simulink model "Kirov_physics"  (R2024b)
settings: Solver=FixedStepDiscrete  StartTime=0.0  StopTime=inf  FixedStep=dt  RelTol=1e-3
undefined symbols (not defined in the file): accel_O, airspeed_bp, alpha_B, alpha_bp, alphaFull, alphaOff, b, battery_capacity_bp, battery_current_bp, battery_initial_capacity_mAh, battery_voltage_table, beta_bp, betaFull, betaOff, brake, brakes, c, channels, CLa, Clb, Clp, CLq, Clr, Cma, Cmq, Cnb, Cnp, Cnr, current_table, DiscIntNeverNeededParam, dt, ELEV_bp, elevator, f, flap, flaps, FLAPS_bp, gear, heightFadeStart, heightOff, hgt_0, Inertia_body, Inertia_load, kInduced, L_aileron, L_throttle, LAILE_bp, lat_0, lon_0, M_aile, M_body, M_elev, M_flap, M_front_gear, M_load, M_main_gear, M_prop, M_rudd, M_spoiler, minWingHeight ... (+36)
libraries: sm_lib x673, simulink x58, nesl_utility x51, simulink_extras x24, uavmavlinklib x12, instrumentlib x4, vrlib x3, aerolibfltsims x3, sharedtransform x3, eeGeneralControl x2, aerolibutil x2, AP_Connector x2
(part 4 of 6)

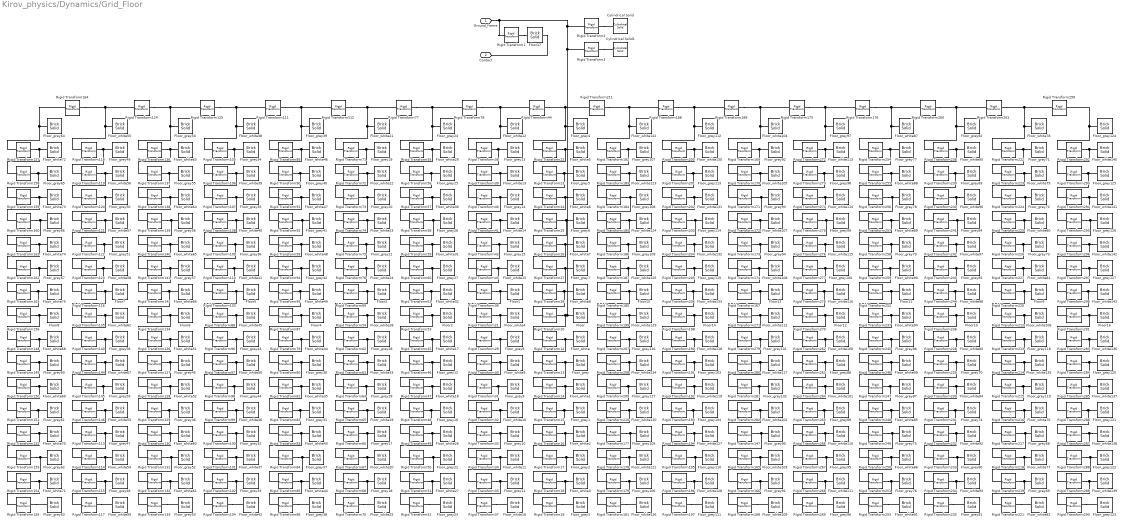
== system Kirov_physics/Dynamics/Grid_Floor ==
  Cylindrical Solid : sm_lib/Body Elements/Cylindrical Solid  CylinderRadius=0.2  CylinderRadiusUnits=m  CylinderLength=5  CylinderLengthUnits=m  ExportEntireGeometry=off  InertiaType=CalculateFromGeometry  BasedOnType=Density  Density=1000  DensityUnits=kg/m^3  Mass=1  MassUnits=kg  CenterOfMass=[0 0 0]  CenterOfMassUnits=m  MomentsOfInertia=[1 1 1]  MomentsOfInertiaUnits=kg*m^2  ProductsOfInertia=[0 0 0]  ProductsOfInertiaUnits=kg*m^2  GraphicType=FromGeometry  MarkerShape=Sphere  MarkerSize=10  GraphicVisPropType=SimpleVisualProperties  GraphicDiffuseColor=[1 0 0]  GraphicOpacity=1  GraphicSpecularColor=[0.5 0.5 0.5 1.0]  GraphicAmbientColor=[0.15 0.15 0.15 1.0]  GraphicEmissiveColor=[0.0 0.0 0.0 1.0]  GraphicShininess=75  DoExposeReferenceFrame=on  SerializedFrames=<Frames/>
  Cylindrical Solid1 : sm_lib/Body Elements/Cylindrical Solid  CylinderRadius=0.2  CylinderRadiusUnits=m  CylinderLength=5  CylinderLengthUnits=m  ExportEntireGeometry=off  InertiaType=CalculateFromGeometry  BasedOnType=Density  Density=1000  DensityUnits=kg/m^3  Mass=1  MassUnits=kg  CenterOfMass=[0 0 0]  CenterOfMassUnits=m  MomentsOfInertia=[1 1 1]  MomentsOfInertiaUnits=kg*m^2  ProductsOfInertia=[0 0 0]  ProductsOfInertiaUnits=kg*m^2  GraphicType=FromGeometry  MarkerShape=Sphere  MarkerSize=10  GraphicVisPropType=SimpleVisualProperties  GraphicDiffuseColor=[1 0 0]  GraphicOpacity=1  GraphicSpecularColor=[0.5 0.5 0.5 1.0]  GraphicAmbientColor=[0.15 0.15 0.15 1.0]  GraphicEmissiveColor=[0.0 0.0 0.0 1.0]  GraphicShininess=75  DoExposeReferenceFrame=on  SerializedFrames=<Frames/>
  Floor{,1..16} (17 alike) : sm_lib/Body Elements/Brick Solid  BrickDimensions=[10 10 0.1]  BrickDimensionsUnits=m  ExportEntireGeometry=off  InertiaType=PointMass  BasedOnType=Density  Density=1000  DensityUnits=kg/m^3  Mass=100  MassUnits=kg  CenterOfMass=[0 0 0]  CenterOfMassUnits=m  MomentsOfInertia=[1 1 1]  MomentsOfInertiaUnits=kg*m^2  ProductsOfInertia=[0 0 0]  ProductsOfInertiaUnits=kg*m^2  GraphicType=FromGeometry  MarkerShape=Sphere  MarkerSize=10  GraphicVisPropType=SimpleVisualProperties  GraphicDiffuseColor=[0.651 0.651 0.651]  GraphicOpacity=1  GraphicSpecularColor=[0.5 0.5 0.5 1.0]  GraphicAmbientColor=[0.15 0.15 0.15 1.0]  GraphicEmissiveColor=[0.0 0.0 0.0 1.0]  GraphicShininess=75  DoExposeReferenceFrame=on  SerializedFrames=<Frames/>
  Floor17 : sm_lib/Body Elements/Brick Solid  BrickDimensions=[2000 2000 0.1]  BrickDimensionsUnits=m  ExportEntireGeometry=on  InertiaType=PointMass  BasedOnType=Density  Density=1000  DensityUnits=kg/m^3  Mass=100  MassUnits=kg  CenterOfMass=[0 0 0]  CenterOfMassUnits=m  MomentsOfInertia=[1 1 1]  MomentsOfInertiaUnits=kg*m^2  ProductsOfInertia=[0 0 0]  ProductsOfInertiaUnits=kg*m^2  GraphicType=FromGeometry  MarkerShape=Sphere  MarkerSize=10  GraphicVisPropType=SimpleVisualProperties  GraphicDiffuseColor=[0.651 0.651 0.651]  GraphicOpacity=1  GraphicSpecularColor=[0.5 0.5 0.5 1.0]  GraphicAmbientColor=[0.15 0.15 0.15 1.0]  GraphicEmissiveColor=[0.0 0.0 0.0 1.0]  GraphicShininess=75  DoExposeReferenceFrame=on  SerializedFrames=<Frames/>
  Floor_grey{,1..127} (128 alike) : sm_lib/Body Elements/Brick Solid  BrickDimensions=[10 10 0.1]  BrickDimensionsUnits=m  ExportEntireGeometry=off  InertiaType=PointMass  BasedOnType=Density  Density=1000  DensityUnits=kg/m^3  Mass=100  MassUnits=kg  CenterOfMass=[0 0 0]  CenterOfMassUnits=m  MomentsOfInertia=[1 1 1]  MomentsOfInertiaUnits=kg*m^2  ProductsOfInertia=[0 0 0]  ProductsOfInertiaUnits=kg*m^2  GraphicType=FromGeometry  MarkerShape=Sphere  MarkerSize=10  GraphicVisPropType=SimpleVisualProperties  GraphicDiffuseColor=[0.651 0.651 0.651]  GraphicOpacity=1  GraphicSpecularColor=[0.5 0.5 0.5 1.0]  GraphicAmbientColor=[0.15 0.15 0.15 1.0]  GraphicEmissiveColor=[0.0 0.0 0.0 1.0]  GraphicShininess=75  DoExposeReferenceFrame=on  SerializedFrames=<Frames/>
  Floor_white{,1..143} (144 alike) : sm_lib/Body Elements/Brick Solid  BrickDimensions=[10 10 0.1]  BrickDimensionsUnits=m  ExportEntireGeometry=off  InertiaType=PointMass  BasedOnType=Density  Density=1000  DensityUnits=kg/m^3  Mass=100  MassUnits=kg  CenterOfMass=[0 0 0]  CenterOfMassUnits=m  MomentsOfInertia=[1 1 1]  MomentsOfInertiaUnits=kg*m^2  ProductsOfInertia=[0 0 0]  ProductsOfInertiaUnits=kg*m^2  GraphicType=FromGeometry  MarkerShape=Sphere  MarkerSize=10  GraphicVisPropType=SimpleVisualProperties  GraphicDiffuseColor=[1 1 1]  GraphicOpacity=1  GraphicSpecularColor=[0.5 0.5 0.5 1.0]  GraphicAmbientColor=[0.15 0.15 0.15 1.0]  GraphicEmissiveColor=[0.0 0.0 0.0 1.0]  GraphicShininess=75  DoExposeReferenceFrame=on  SerializedFrames=<Frames/>
  Rigid Transform1 : sm_lib/Frames and Transforms/Rigid Transform  RotationMethod=None  FollAlignAxisA=+X  BaseAlignAxisA=+Y  FollAlignAxisB=+Y  BaseAlignAxisB=+Z  RotationStandardAxis=+Z  RotationAngle=0  RotationAngleUnits=deg  RotationArbitraryAxis=[0 0 1]  RotationSequenceAxes=FollowerAxes  RotationSequence=XYX  RotationSequenceAngles=[0 0 0]  RotationSequenceAnglesUnits=deg  RotationMatrix=[1 0 0;0 1 0;0 0 1]  Quaternion=[1 0 0 0]  TranslationMethod=Cartesian  TranslationCartesianOffset=[0 0 0.005]  TranslationCartesianOffsetUnits=m  TranslationStandardAxis=+Z  TranslationStandardOffset=0  TranslationStandardOffsetUnits=m  TranslationROffset=0  TranslationROffsetUnits=m  TranslationThetaOffset=0  TranslationThetaOffsetUnits=deg  TranslationZOffset=0  TranslationZOffsetUnits=m
  Rigid Transform{12..43,45..76,79..110,113..123,126..163,165..174,177..187,190..210,212..259,262..298} (272 alike) : sm_lib/Frames and Transforms/Rigid Transform  RotationMethod=None  FollAlignAxisA=+X  BaseAlignAxisA=+Y  FollAlignAxisB=+Y  BaseAlignAxisB=+Z  RotationStandardAxis=+Z  RotationAngle=0  RotationAngleUnits=deg  RotationArbitraryAxis=[0 0 1]  RotationSequenceAxes=FollowerAxes  RotationSequence=XYX  RotationSequenceAngles=[0 0 0]  RotationSequenceAnglesUnits=deg  RotationMatrix=[1 0 0;0 1 0;0 0 1]  Quaternion=[1 0 0 0]  TranslationMethod=Cartesian  TranslationCartesianOffset=[10 0 0]  TranslationCartesianOffsetUnits=m  TranslationStandardAxis=+Z  TranslationStandardOffset=0  TranslationStandardOffsetUnits=m  TranslationROffset=0  TranslationROffsetUnits=m  TranslationThetaOffset=0  TranslationThetaOffsetUnits=deg  TranslationZOffset=0  TranslationZOffsetUnits=m
  Rigid Transform{44,77..78,111..112,124..125,164,175..176,188..189,211,260..261,299} (16 alike) : sm_lib/Frames and Transforms/Rigid Transform  RotationMethod=None  FollAlignAxisA=+X  BaseAlignAxisA=+Y  FollAlignAxisB=+Y  BaseAlignAxisB=+Z  RotationStandardAxis=+Z  RotationAngle=0  RotationAngleUnits=deg  RotationArbitraryAxis=[0 0 1]  RotationSequenceAxes=FollowerAxes  RotationSequence=XYX  RotationSequenceAngles=[0 0 0]  RotationSequenceAnglesUnits=deg  RotationMatrix=[1 0 0;0 1 0;0 0 1]  Quaternion=[1 0 0 0]  TranslationMethod=Cartesian  TranslationCartesianOffset=[0 10 0]  TranslationCartesianOffsetUnits=m  TranslationStandardAxis=+Z  TranslationStandardOffset=0  TranslationStandardOffsetUnits=m  TranslationROffset=0  TranslationROffsetUnits=m  TranslationThetaOffset=0  TranslationThetaOffsetUnits=deg  TranslationZOffset=0  TranslationZOffsetUnits=m
  Rigid Transform2 : sm_lib/Frames and Transforms/Rigid Transform  RotationMethod=None  FollAlignAxisA=+X  BaseAlignAxisA=+Y  FollAlignAxisB=+Y  BaseAlignAxisB=+Z  RotationStandardAxis=+Z  RotationAngle=0  RotationAngleUnits=deg  RotationArbitraryAxis=[0 0 1]  RotationSequenceAxes=FollowerAxes  RotationSequence=XYX  RotationSequenceAngles=[0 0 0]  RotationSequenceAnglesUnits=deg  RotationMatrix=[1 0 0;0 1 0;0 0 1]  Quaternion=[1 0 0 0]  TranslationMethod=Cartesian  TranslationCartesianOffset=[50 20 -2.5]  TranslationCartesianOffsetUnits=m  TranslationStandardAxis=+Z  TranslationStandardOffset=0  TranslationStandardOffsetUnits=m  TranslationROffset=0  TranslationROffsetUnits=m  TranslationThetaOffset=0  TranslationThetaOffsetUnits=deg  TranslationZOffset=0  TranslationZOffsetUnits=m
  Rigid Transform3 : sm_lib/Frames and Transforms/Rigid Transform  RotationMethod=None  FollAlignAxisA=+X  BaseAlignAxisA=+Y  FollAlignAxisB=+Y  BaseAlignAxisB=+Z  RotationStandardAxis=+Z  RotationAngle=0  RotationAngleUnits=deg  RotationArbitraryAxis=[0 0 1]  RotationSequenceAxes=FollowerAxes  RotationSequence=XYX  RotationSequenceAngles=[0 0 0]  RotationSequenceAnglesUnits=deg  RotationMatrix=[1 0 0;0 1 0;0 0 1]  Quaternion=[1 0 0 0]  TranslationMethod=Cartesian  TranslationCartesianOffset=[-50 20 -2.5]  TranslationCartesianOffsetUnits=m  TranslationStandardAxis=+Z  TranslationStandardOffset=0  TranslationStandardOffsetUnits=m  TranslationROffset=0  TranslationROffsetUnits=m  TranslationThetaOffset=0  TranslationThetaOffsetUnits=deg  TranslationZOffset=0  TranslationZOffsetUnits=m
  Ground_frame : PMIOPort  Side=Left
  Contact : PMIOPort  Port=2  Side=Right
  connections:
  Rigid Transform158/RConn1 -- Rigid Transform159/LConn1 -- Floor_grey65/RConn1
  Rigid Transform156/LConn1 -- Rigid Transform163/RConn1 -- Floor_white75/RConn1
  Rigid Transform168/RConn1 -- Floor_white109/RConn1
  Floor_white120/RConn1 -- Rigid Transform177/LConn1 -- Rigid Transform210/RConn1
  Rigid Transform198/LConn1 -- Rigid Transform206/RConn1 -- Floor_white133/RConn1
  Floor_white85/RConn1 -- Rigid Transform249/LConn1 -- Rigid Transform248/RConn1
  Rigid Transform244/LConn1 -- Rigid Transform243/RConn1 -- Floor_grey85/RConn1
  Rigid Transform245/RConn1 -- Rigid Transform246/LConn1 -- Floor_grey86/RConn1
  Floor_white122/RConn1 -- Rigid Transform211/RConn1 -- Rigid Transform188/LConn1 -- Rigid Transform182/LConn1
  Rigid Transform241/RConn1 -- Rigid Transform242/LConn1 -- Floor_grey84/RConn1
  Rigid Transform284/RConn1 -- Rigid Transform285/LConn1 -- Floor_grey120/RConn1
  Floor8/RConn1 -- Rigid Transform156/RConn1 -- Rigid Transform148/LConn1
  Floor_white93/RConn1 -- Rigid Transform235/LConn1 -- Rigid Transform234/RConn1
  Rigid Transform180/RConn1 -- Floor15/RConn1 -- Rigid Transform199/LConn1
  Rigid Transform282/LConn1 -- Rigid Transform281/RConn1 -- Floor_grey102/RConn1
  Rigid Transform127/RConn1 -- Rigid Transform128/LConn1 -- Floor_grey45/RConn1
  Rigid Transform243/LConn1 -- Floor_white97/RConn1 -- Rigid Transform242/RConn1
  Rigid Transform160/RConn1 -- Rigid Transform161/LConn1 -- Floor_grey66/RConn1
  Rigid Transform133/LConn1 -- Floor_white61/RConn1 -- Rigid Transform132/RConn1
  Rigid Transform257/LConn1 -- Rigid Transform256/RConn1 -- Floor_grey78/RConn1
  Rigid Transform123/LConn1 -- Rigid Transform122/RConn1 -- Floor_grey51/RConn1
  Rigid Transform295/LConn1 -- Floor_white141/RConn1 -- Rigid Transform294/RConn1
  Rigid Transform184/LConn1 -- Floor_white123/RConn1 -- Rigid Transform183/RConn1
  Rigid Transform120/RConn1 -- Rigid Transform121/LConn1 -- Floor_grey50/RConn1
  Rigid Transform226/LConn1 -- Floor_white80/RConn1 -- Rigid Transform225/RConn1
  Rigid Transform224/RConn1 -- Rigid Transform225/LConn1 -- Floor_grey72/RConn1
  Floor_white131/RConn1 -- Rigid Transform203/LConn1 -- Rigid Transform202/RConn1
  Rigid Transform152/LConn1 -- Rigid Transform151/RConn1 -- Floor_grey61/RConn1
  Floor_white65/RConn1 -- Rigid Transform141/LConn1 -- Rigid Transform140/RConn1
  Rigid Transform144/RConn1 -- Rigid Transform145/LConn1 -- Floor_white67/RConn1
  Rigid Transform197/RConn1 -- Floor_grey111/RConn1
  Rigid Transform179/LConn1 -- Floor_white121/RConn1 -- Rigid Transform178/RConn1
  Rigid Transform122/LConn1 -- Floor_white57/RConn1 -- Rigid Transform121/RConn1
  Rigid Transform52/LConn1 -- Floor_white27/RConn1 -- Rigid Transform51/RConn1
  Rigid Transform58/LConn1 -- Floor_white30/RConn1 -- Rigid Transform57/RConn1
  Rigid Transform283/RConn1 -- Rigid Transform284/LConn1 -- Floor_white136/RConn1
  Rigid Transform57/LConn1 -- Rigid Transform56/RConn1 -- Floor_grey25/RConn1
  Floor_white105/RConn1 -- Rigid Transform171/LConn1 -- Rigid Transform170/RConn1
  Rigid Transform201/LConn1 -- Rigid Transform200/RConn1 -- Floor_white130/RConn1
  Rigid Transform150/RConn1 -- Rigid Transform151/LConn1 -- Floor_white69/RConn1
  Rigid Transform181/RConn1 -- Floor_white126/RConn1
  Rigid Transform158/LConn1 -- Rigid Transform157/RConn1 -- Floor_white72/RConn1
  Rigid Transform256/LConn1 -- Floor_white88/RConn1 -- Rigid Transform255/RConn1
  Floor_white26/RConn1 -- Rigid Transform50/LConn1 -- Rigid Transform49/RConn1
  Rigid Transform163/LConn1 -- Rigid Transform162/RConn1 -- Floor_grey67/RConn1
  Rigid Transform70/RConn1 -- Floor_white25/RConn1
  Rigid Transform147/LConn1 -- Floor_white102/RConn1 -- Rigid Transform282/RConn1
  Rigid Transform201/RConn1 -- Rigid Transform202/LConn1 -- Floor_grey113/RConn1
  Rigid Transform277/RConn1 -- Rigid Transform278/LConn1 -- Floor_grey100/RConn1
  Rigid Transform175/RConn1 -- Rigid Transform176/LConn1 -- Rigid Transform272/LConn1 -- Floor_grey97/RConn1
  Rigid Transform211/LConn1 -- Rigid Transform44/RConn1 -- Floor_grey4/RConn1 -- Rigid Transform22/LConn1
  Rigid Transform196/LConn1 -- Rigid Transform195/RConn1 -- Floor_grey110/RConn1
  Rigid Transform183/LConn1 -- Rigid Transform182/RConn1 -- Floor_grey107/RConn1
  Rigid Transform136/RConn1 -- Rigid Transform137/LConn1 -- Floor_white63/RConn1
  Rigid Transform23/RConn1 -- Rigid Transform24/LConn1 -- Floor_grey5/RConn1
  Rigid Transform23/LConn1 -- Rigid Transform22/RConn1 -- Floor_white5/RConn1
  Rigid Transform14/LConn1 -- Rigid Transform13/RConn1 -- Floor_grey/RConn1
  Rigid Transform239/LConn1 -- Rigid Transform238/RConn1 -- Floor_white95/RConn1
  Rigid Transform194/LConn1 -- Rigid Transform193/RConn1 -- Floor_grey104/RConn1
  Rigid Transform138/LConn1 -- Rigid Transform137/RConn1 -- Floor_grey55/RConn1
  Rigid Transform191/LConn1 -- Rigid Transform190/RConn1 -- Floor_white118/RConn1
  Rigid Transform27/LConn1 -- Floor_white7/RConn1 -- Rigid Transform26/RConn1
  Rigid Transform269/RConn1 -- Floor_grey96/RConn1
  Floor_white60/RConn1 -- Rigid Transform131/LConn1 -- Rigid Transform130/RConn1
  Rigid Transform237/RConn1 -- Rigid Transform245/LConn1 -- Floor_white94/RConn1
  Rigid Transform43/RConn1 -- Rigid Transform36/LConn1 -- Floor_white15/RConn1
  Rigid Transform45/RConn1 -- Rigid Transform46/LConn1 -- Floor_white17/RConn1
  Rigid Transform13/LConn1 -- Rigid Transform12/RConn1 -- Floor_white/RConn1
  Rigid Transform78/RConn1 -- Rigid Transform38/LConn1 -- Floor_white12/RConn1 -- Rigid Transform44/LConn1
  Rigid Transform220/LConn1 -- Rigid Transform227/RConn1 -- Floor_white81/RConn1
  Rigid Transform134/RConn1 -- Floor6/RConn1 -- Rigid Transform126/LConn1
  Rigid Transform259/RConn1 -- Rigid Transform252/LConn1 -- Floor_white90/RConn1
  Floor_white14/RConn1 -- Rigid Transform42/LConn1 -- Rigid Transform41/RConn1
  Rigid Transform143/LConn1 -- Rigid Transform135/RConn1 -- Floor_white62/RConn1
  Rigid Transform294/LConn1 -- Rigid Transform293/RConn1 -- Floor_grey125/RConn1
  Rigid Transform279/LConn1 -- Rigid Transform271/RConn1 -- Floor_white112/RConn1
  Rigid Transform133/RConn1 -- Floor_grey53/RConn1
  Rigid Transform144/LConn1 -- Rigid Transform143/RConn1 -- Floor_grey58/RConn1
  Rigid Transform33/RConn1 -- Rigid Transform34/LConn1 -- Floor_grey10/RConn1
  Rigid Transform169/RConn1 -- Rigid Transform170/LConn1 -- Floor_grey92/RConn1
  Rigid Transform114/LConn1 -- Rigid Transform113/RConn1 -- Floor_grey47/RConn1
  Rigid Transform17/LConn1 -- Floor_white2/RConn1 -- Rigid Transform16/RConn1
  Rigid Transform164/LConn1 -- Floor_grey64/RConn1 -- Rigid Transform157/LConn1
  Rigid Transform25/RConn1 -- Rigid Transform26/LConn1 -- Floor_grey6/RConn1
  Rigid Transform209/LConn1 -- Rigid Transform208/RConn1 -- Floor_white134/RConn1
  Rigid Transform21/RConn1 -- Rigid Transform29/LConn1 -- Floor_white4/RConn1
  Rigid Transform14/RConn1 -- Rigid Transform15/LConn1 -- Floor_white1/RConn1
  Floor_white128/RConn1 -- Rigid Transform197/LConn1 -- Rigid Transform196/RConn1
  Rigid Transform140/LConn1 -- Rigid Transform139/RConn1 -- Floor_grey56/RConn1
  Rigid Transform42/RConn1 -- Rigid Transform43/LConn1 -- Floor_grey15/RConn1
  Floor_white10/RConn1 -- Rigid Transform33/LConn1 -- Rigid Transform32/RConn1
  Rigid Transform230/RConn1 -- Rigid Transform231/LConn1 -- Floor_white84/RConn1
  Floor_white142/RConn1 -- Rigid Transform297/LConn1 -- Rigid Transform296/RConn1
  Rigid Transform116/LConn1 -- Rigid Transform123/RConn1 -- Floor_white58/RConn1
  Rigid Transform67/LConn1 -- Rigid Transform66/RConn1 -- Floor_grey17/RConn1
  Rigid Transform192/RConn1 -- Rigid Transform193/LConn1 -- Floor_white119/RConn1
  Floor10/RConn1 -- Rigid Transform236/RConn1 -- Rigid Transform228/LConn1
  Rigid Transform213/LConn1 -- Rigid Transform212/RConn1 -- Floor_white106/RConn1
  Floor_white138/RConn1 -- Rigid Transform288/LConn1 -- Rigid Transform287/RConn1
  Floor_white73/RConn1 -- Rigid Transform160/LConn1 -- Rigid Transform159/RConn1
  Rigid Transform37/LConn1 -- Rigid Transform35/RConn1 -- Floor_grey11/RConn1
  Rigid Transform19/RConn1 -- Floor_grey3/RConn1
  Floor_white3/RConn1 -- Rigid Transform19/LConn1 -- Rigid Transform18/RConn1
  Rigid Transform139/LConn1 -- Floor_white64/RConn1 -- Rigid Transform138/RConn1
  Ground_frame/RConn1 -- Rigid Transform1/LConn1 -- Rigid Transform2/LConn1 -- Rigid Transform3/LConn1 -- Floor/RConn1 -- Rigid Transform20/RConn1 -- Rigid Transform12/LConn1
  Rigid Transform46/RConn1 -- Rigid Transform47/LConn1 -- Floor_grey12/RConn1
  Rigid Transform50/RConn1 -- Rigid Transform51/LConn1 -- Floor_grey22/RConn1
  Floor3/RConn1 -- Rigid Transform69/RConn1 -- Rigid Transform54/LConn1
  Rigid Transform31/RConn1 -- Rigid Transform32/LConn1 -- Floor_grey9/RConn1
  Rigid Transform60/RConn1 -- Rigid Transform61/LConn1 -- Floor_grey27/RConn1
  Rigid Transform232/LConn1 -- Rigid Transform231/RConn1 -- Floor_grey74/RConn1
  Rigid Transform280/LConn1 -- Rigid Transform279/RConn1 -- Floor_grey101/RConn1
  Rigid Transform219/RConn1 -- Rigid Transform221/LConn1 -- Floor_grey69/RConn1
  Rigid Transform298/RConn1 -- Rigid Transform291/LConn1 -- Floor_white143/RConn1
  Rigid Transform48/RConn1 -- Rigid Transform49/LConn1 -- Floor_grey16/RConn1
  Rigid Transform154/LConn1 -- Rigid Transform153/RConn1 -- Floor_grey62/RConn1
  Rigid Transform100/RConn1 -- Rigid Transform101/LConn1 -- Floor_grey32/RConn1
  Rigid Transform263/RConn1 -- Rigid Transform264/LConn1 -- Floor_grey88/RConn1
  Rigid Transform235/RConn1 -- Floor_grey81/RConn1
  Rigid Transform166/RConn1 -- Rigid Transform168/LConn1 -- Floor_grey91/RConn1
  Rigid Transform269/LConn1 -- Floor_white111/RConn1 -- Rigid Transform268/RConn1
  Floor_white20/RConn1 -- Rigid Transform68/LConn1 -- Rigid Transform67/RConn1
  Rigid Transform288/RConn1 -- Rigid Transform289/LConn1 -- Floor_grey122/RConn1
  Rigid Transform98/LConn1 -- Rigid Transform97/RConn1 -- Floor_white50/RConn1
  Rigid Transform62/LConn1 -- Rigid Transform54/RConn1 -- Floor_white28/RConn1
  Rigid Transform292/RConn1 -- Rigid Transform293/LConn1 -- Floor_white140/RConn1
  Floor14/RConn1 -- Rigid Transform198/RConn1 -- Rigid Transform190/LConn1
  Rigid Transform98/RConn1 -- Rigid Transform99/LConn1 -- Floor_grey44/RConn1
  Rigid Transform189/LConn1 -- Rigid Transform188/RConn1 -- Floor_grey112/RConn1 -- Rigid Transform200/LConn1
  Rigid Transform272/RConn1 -- Rigid Transform273/LConn1 -- Floor_white113/RConn1
  Rigid Transform65/LConn1 -- Rigid Transform64/RConn1 -- Floor_grey29/RConn1
  Rigid Transform131/RConn1 -- Rigid Transform132/LConn1 -- Floor_grey52/RConn1
  Rigid Transform125/RConn1 -- Rigid Transform111/LConn1 -- Rigid Transform105/LConn1 -- Floor_white38/RConn1
  Floor_white87/RConn1 -- Rigid Transform260/LConn1 -- Rigid Transform176/RConn1 -- Rigid Transform254/LConn1
  Rigid Transform169/LConn1 -- Rigid Transform189/RConn1 -- Rigid Transform175/LConn1 -- Floor_white104/RConn1
  Floor_white36/RConn1 -- Rigid Transform100/LConn1 -- Rigid Transform99/RConn1
  Rigid Transform95/LConn1 -- Rigid Transform94/RConn1 -- Floor_grey42/RConn1
  Rigid Transform149/LConn1 -- Rigid Transform148/RConn1 -- Floor_white68/RConn1
  Rigid Transform142/RConn1 -- Rigid Transform134/LConn1 -- Floor_white66/RConn1
  Rigid Transform18/LConn1 -- Rigid Transform17/RConn1 -- Floor_grey2/RConn1
  Rigid Transform41/LConn1 -- Rigid Transform40/RConn1 -- Floor_grey14/RConn1
  Floor13/RConn1 -- Rigid Transform167/RConn1 -- Rigid Transform271/LConn1
  Rigid Transform251/LConn1 -- Floor_white86/RConn1 -- Rigid Transform250/RConn1
  Rigid Transform113/LConn1 -- Floor_white53/RConn1 -- Rigid Transform146/RConn1
  Floor_white115/RConn1 -- Rigid Transform277/LConn1 -- Rigid Transform276/RConn1
  Rigid Transform181/LConn1 -- Rigid Transform179/RConn1 -- Floor_grey106/RConn1
  Floor_white31/RConn1 -- Rigid Transform60/LConn1 -- Rigid Transform59/RConn1
  Floor7/RConn1 -- Rigid Transform116/RConn1 -- Rigid Transform135/LConn1
  Floor_white56/RConn1 -- Rigid Transform120/LConn1 -- Rigid Transform119/RConn1
  Rigid Transform236/LConn1 -- Rigid Transform244/RConn1 -- Floor_white98/RConn1
  Floor_white79/RConn1 -- Rigid Transform224/LConn1 -- Rigid Transform223/RConn1
  Rigid Transform29/RConn1 -- Rigid Transform30/LConn1 -- Floor_grey8/RConn1
  Rigid Transform16/LConn1 -- Rigid Transform15/RConn1 -- Floor_grey1/RConn1
  Rigid Transform270/RConn1 -- Floor12/RConn1 -- Rigid Transform262/LConn1
  Rigid Transform174/LConn1 -- Rigid Transform173/RConn1 -- Floor_grey94/RConn1
  Rigid Transform92/RConn1 -- Rigid Transform93/LConn1 -- Floor_grey41/RConn1
  Rigid Transform286/RConn1 -- Rigid Transform287/LConn1 -- Floor_grey121/RConn1
  Rigid Transform55/RConn1 -- Rigid Transform56/LConn1 -- Floor_white29/RConn1
  Rigid Transform94/LConn1 -- Floor_white48/RConn1 -- Rigid Transform93/RConn1
  Rigid Transform275/LConn1 -- Floor_white114/RConn1 -- Rigid Transform274/RConn1
  Floor_white47/RConn1 -- Rigid Transform92/LConn1 -- Rigid Transform91/RConn1
  Rigid Transform117/RConn1 -- Floor_white59/RConn1
  Rigid Transform227/LConn1 -- Rigid Transform226/RConn1 -- Floor_grey73/RConn1
  Rigid Transform207/RConn1 -- Rigid Transform208/LConn1 -- Floor_grey116/RConn1
  Floor_white44/RConn1 -- Rigid Transform86/LConn1 -- Rigid Transform85/RConn1
  Rigid Transform63/LConn1 -- Rigid Transform62/RConn1 -- Floor_grey28/RConn1
  Rigid Transform78/LConn1 -- Rigid Transform77/RConn1 -- Rigid Transform55/LConn1 -- Floor_grey24/RConn1
  Rigid Transform299/RConn1 -- Rigid Transform292/LConn1 -- Floor_grey124/RConn1
  Rigid Transform229/LConn1 -- Rigid Transform228/RConn1 -- Floor_white83/RConn1
  Rigid Transform90/RConn1 -- Rigid Transform91/LConn1 -- Floor_grey40/RConn1
  Rigid Transform253/LConn1 -- Rigid Transform251/RConn1 -- Floor_grey76/RConn1
  Rigid Transform141/RConn1 -- Rigid Transform142/LConn1 -- Floor_grey57/RConn1
  Rigid Transform286/LConn1 -- Rigid Transform285/RConn1 -- Floor_white137/RConn1
  Rigid Transform262/RConn1 -- Rigid Transform263/LConn1 -- Floor_white100/RConn1
  Rigid Transform129/RConn1 -- Rigid Transform130/LConn1 -- Floor_grey46/RConn1
  Rigid Transform69/LConn1 -- Rigid Transform76/RConn1 -- Floor_white24/RConn1
  Rigid Transform217/LConn1 -- Floor_white76/RConn1 -- Rigid Transform216/RConn1
  Rigid Transform233/LConn1 -- Floor_white92/RConn1 -- Rigid Transform232/RConn1
  Floor_white103/RConn1 -- Rigid Transform166/LConn1 -- Rigid Transform165/RConn1
  Rigid Transform234/LConn1 -- Rigid Transform233/RConn1 -- Floor_grey80/RConn1
  Rigid Transform115/RConn1 -- Rigid Transform117/LConn1 -- Floor_grey48/RConn1
  Rigid Transform173/LConn1 -- Floor_white107/RConn1 -- Rigid Transform172/RConn1
  Rigid Transform214/LConn1 -- Rigid Transform213/RConn1 -- Floor_grey118/RConn1
  Rigid Transform36/RConn1 -- Floor1/RConn1 -- Rigid Transform21/LConn1
  Floor_white54/RConn1 -- Rigid Transform115/LConn1 -- Rigid Transform114/RConn1
  Rigid Transform146/LConn1 -- Rigid Transform145/RConn1 -- Floor_grey59/RConn1
  Rigid Transform247/LConn1 -- Rigid Transform246/RConn1 -- Floor_white99/RConn1
  Rigid Transform71/RConn1 -- Rigid Transform72/LConn1 -- Floor_grey19/RConn1
  Rigid Transform103/RConn1 -- Floor5/RConn1 -- Rigid Transform88/LConn1
  Rigid Transform153/LConn1 -- Floor_white70/RConn1 -- Rigid Transform152/RConn1
  Rigid Transform81/LConn1 -- Rigid Transform80/RConn1 -- Floor_grey30/RConn1
  Rigid Transform37/RConn1 -- Floor_white16/RConn1
  Rigid Transform35/LConn1 -- Floor_white11/RConn1 -- Rigid Transform34/RConn1
  Rigid Transform150/LConn1 -- Rigid Transform149/RConn1 -- Floor_grey60/RConn1
  Floor_white40/RConn1 -- Rigid Transform109/LConn1 -- Rigid Transform108/RConn1
  Rigid Transform102/LConn1 -- Floor_white37/RConn1 -- Rigid Transform101/RConn1
  Rigid Transform31/LConn1 -- Rigid Transform30/RConn1 -- Floor_white9/RConn1
  Rigid Transform52/RConn1 -- Floor_grey23/RConn1
  Rigid Transform205/LConn1 -- Floor_white132/RConn1 -- Rigid Transform204/RConn1
  Rigid Transform278/RConn1 -- Rigid Transform270/LConn1 -- Floor_white116/RConn1
  Rigid Transform276/LConn1 -- Rigid Transform275/RConn1 -- Floor_grey99/RConn1
  Rigid Transform104/LConn1 -- Rigid Transform102/RConn1 -- Floor_grey33/RConn1
  Rigid Transform155/RConn1 -- Floor_grey63/RConn1
  Rigid Transform89/LConn1 -- Rigid Transform112/LConn1 -- Rigid Transform111/RConn1 -- Floor_grey39/RConn1
  Rigid Transform255/LConn1 -- Rigid Transform254/RConn1 -- Floor_grey77/RConn1
  Rigid Transform177/RConn1 -- Rigid Transform178/LConn1 -- Floor_grey105/RConn1
  Rigid Transform83/LConn1 -- Rigid Transform82/RConn1 -- Floor_grey31/RConn1
  Rigid Transform186/RConn1 -- Rigid Transform187/LConn1 -- Floor_grey109/RConn1
  Rigid Transform39/LConn1 -- Rigid Transform38/RConn1 -- Floor_grey13/RConn1
  Rigid Transform107/LConn1 -- Floor_white39/RConn1 -- Rigid Transform106/RConn1
  Rigid Transform73/RConn1 -- Rigid Transform74/LConn1 -- Floor_grey20/RConn1
  Floor_white6/RConn1 -- Rigid Transform25/LConn1 -- Rigid Transform24/RConn1
  Rigid Transform68/RConn1 -- Rigid Transform70/LConn1 -- Floor_grey18/RConn1
  Rigid Transform104/RConn1 -- Floor_white42/RConn1
  Rigid Transform63/RConn1 -- Rigid Transform64/LConn1 -- Floor_white33/RConn1
  Rigid Transform40/LConn1 -- Floor_white13/RConn1 -- Rigid Transform39/RConn1
  Floor_white77/RConn1 -- Rigid Transform219/LConn1 -- Rigid Transform218/RConn1
  Rigid Transform165/LConn1 -- Rigid Transform147/RConn1 -- Floor_grey90/RConn1
  Rigid Transform265/RConn1 -- Rigid Transform266/LConn1 -- Floor_grey89/RConn1
  Rigid Transform296/LConn1 -- Rigid Transform295/RConn1 -- Floor_grey126/RConn1
  Rigid Transform106/LConn1 -- Rigid Transform105/RConn1 -- Floor_grey34/RConn1
  Rigid Transform206/LConn1 -- Rigid Transform205/RConn1 -- Floor_grey115/RConn1
  Rigid Transform164/RConn1 -- Rigid Transform124/LConn1 -- Floor_white55/RConn1 -- Rigid Transform118/LConn1
  Rigid Transform66/LConn1 -- Floor_white19/RConn1 -- Rigid Transform65/RConn1
  Rigid Transform124/RConn1 -- Rigid Transform125/LConn1 -- Rigid Transform136/LConn1 -- Floor_grey54/RConn1
  Rigid Transform280/RConn1 -- Rigid Transform281/LConn1 -- Floor_white117/RConn1
  Rigid Transform76/LConn1 -- Rigid Transform75/RConn1 -- Floor_grey21/RConn1
  Rigid Transform218/LConn1 -- Rigid Transform217/RConn1 -- Floor_grey68/RConn1
  Rigid Transform108/LConn1 -- Rigid Transform107/RConn1 -- Floor_grey35/RConn1
  Rigid Transform61/RConn1 -- Rigid Transform53/LConn1 -- Floor_white32/RConn1
  Rigid Transform192/LConn1 -- Rigid Transform191/RConn1 -- Floor_grey103/RConn1
  Rigid Transform20/LConn1 -- Rigid Transform28/RConn1 -- Floor_white8/RConn1
  Rigid Transform214/RConn1 -- Rigid Transform215/LConn1 -- Floor_white135/RConn1
  Floor_white110/RConn1 -- Rigid Transform267/LConn1 -- Rigid Transform266/RConn1
  Rigid Transform59/LConn1 -- Rigid Transform58/RConn1 -- Floor_grey26/RConn1
  Rigid Transform87/LConn1 -- Rigid Transform95/RConn1 -- Floor_white49/RConn1
  Rigid Transform221/RConn1 -- Floor_white82/RConn1
  Rigid Transform86/RConn1 -- Floor_grey38/RConn1
  Floor9/RConn1 -- Rigid Transform220/RConn1 -- Rigid Transform212/LConn1
  Floor_white124/RConn1 -- Rigid Transform186/LConn1 -- Rigid Transform185/RConn1
  Rigid Transform185/LConn1 -- Rigid Transform184/RConn1 -- Floor_grey108/RConn1
  Rigid Transform48/LConn1 -- Rigid Transform47/RConn1 -- Floor_white18/RConn1
  Rigid Transform167/LConn1 -- Rigid Transform174/RConn1 -- Floor_white108/RConn1
  Rigid Transform75/LConn1 -- Floor_white23/RConn1 -- Rigid Transform74/RConn1
  Rigid Transform239/RConn1 -- Rigid Transform240/LConn1 -- Floor_grey83/RConn1
  Rigid Transform203/RConn1 -- Rigid Transform204/LConn1 -- Floor_grey114/RConn1
  Rigid Transform195/LConn1 -- Floor_white127/RConn1 -- Rigid Transform194/RConn1
  Rigid Transform258/RConn1 -- Rigid Transform259/LConn1 -- Floor_grey79/RConn1
  Rigid Transform290/LConn1 -- Floor_white139/RConn1 -- Rigid Transform289/RConn1
  Rigid Transform85/LConn1 -- Rigid Transform84/RConn1 -- Floor_grey37/RConn1
  Rigid Transform249/RConn1 -- Rigid Transform250/LConn1 -- Floor_grey75/RConn1
  Rigid Transform110/RConn1 -- Rigid Transform103/LConn1 -- Floor_white41/RConn1
  Rigid Transform253/RConn1 -- Floor_white91/RConn1
  Rigid Transform162/LConn1 -- Floor_white74/RConn1 -- Rigid Transform161/RConn1
  Rigid Transform216/LConn1 -- Rigid Transform215/RConn1 -- Floor_grey119/RConn1
  Rigid Transform81/RConn1 -- Rigid Transform82/LConn1 -- Floor_white35/RConn1
  Rigid Transform252/RConn1 -- Floor11/RConn1 -- Rigid Transform237/LConn1
  Rigid Transform291/RConn1 -- Floor16/RConn1 -- Rigid Transform283/LConn1
  Rigid Transform187/RConn1 -- Rigid Transform180/LConn1 -- Floor_white125/RConn1
  Rigid Transform84/LConn1 -- Floor_white43/RConn1 -- Rigid Transform83/RConn1
  Rigid Transform129/LConn1 -- Rigid Transform128/RConn1 -- Floor_white52/RConn1
  Rigid Transform238/LConn1 -- Rigid Transform261/LConn1 -- Rigid Transform260/RConn1 -- Floor_grey82/RConn1
  Rigid Transform230/LConn1 -- Rigid Transform229/RConn1 -- Floor_grey70/RConn1
  Floor_white89/RConn1 -- Rigid Transform258/LConn1 -- Rigid Transform257/RConn1
  Floor_white22/RConn1 -- Rigid Transform73/LConn1 -- Rigid Transform72/RConn1
  Rigid Transform222/RConn1 -- Rigid Transform223/LConn1 -- Floor_grey71/RConn1
  Floor_white71/RConn1 -- Rigid Transform155/LConn1 -- Rigid Transform154/RConn1
  Rigid Transform109/RConn1 -- Rigid Transform110/LConn1 -- Floor_grey36/RConn1
  Rigid Transform90/LConn1 -- Rigid Transform89/RConn1 -- Floor_white46/RConn1
  Rigid Transform126/RConn1 -- Rigid Transform127/LConn1 -- Floor_white51/RConn1
  Rigid Transform88/RConn1 -- Rigid Transform96/LConn1 -- Floor_white45/RConn1
  Rigid Transform274/LConn1 -- Rigid Transform273/RConn1 -- Floor_grey98/RConn1
  Rigid Transform267/RConn1 -- Rigid Transform268/LConn1 -- Floor_grey95/RConn1
  Rigid Transform80/LConn1 -- Rigid Transform79/RConn1 -- Floor_white34/RConn1
  Rigid Transform297/RConn1 -- Rigid Transform298/LConn1 -- Floor_grey127/RConn1
  Rigid Transform118/RConn1 -- Rigid Transform119/LConn1 -- Floor_grey49/RConn1
  Rigid Transform53/RConn1 -- Floor2/RConn1 -- Rigid Transform45/LConn1
  Rigid Transform299/LConn1 -- Floor_white78/RConn1 -- Rigid Transform222/LConn1 -- Rigid Transform261/RConn1
  Floor4/RConn1 -- Rigid Transform87/RConn1 -- Rigid Transform79/LConn1
  Rigid Transform247/RConn1 -- Rigid Transform248/LConn1 -- Floor_grey87/RConn1
  Rigid Transform265/LConn1 -- Rigid Transform264/RConn1 -- Floor_white101/RConn1
  Rigid Transform171/RConn1 -- Rigid Transform172/LConn1 -- Floor_grey93/RConn1
  Rigid Transform290/RConn1 -- Floor_grey123/RConn1
  Rigid Transform199/RConn1 -- Rigid Transform207/LConn1 -- Floor_white129/RConn1
  Rigid Transform112/RConn1 -- Floor_white21/RConn1 -- Rigid Transform71/LConn1 -- Rigid Transform77/LConn1
  Floor_white96/RConn1 -- Rigid Transform241/LConn1 -- Rigid Transform240/RConn1
  Rigid Transform209/RConn1 -- Rigid Transform210/LConn1 -- Floor_grey117/RConn1
  Rigid Transform96/RConn1 -- Rigid Transform97/LConn1 -- Floor_grey43/RConn1
  Rigid Transform28/LConn1 -- Rigid Transform27/RConn1 -- Floor_grey7/RConn1
  Floor17/LConn1 -- Contact/RConn1
  Rigid Transform1/RConn1 -- Floor17/RConn1
  Rigid Transform2/RConn1 -- Cylindrical Solid/RConn1
  Rigid Transform3/RConn1 -- Cylindrical Solid1/RConn1

== system Kirov_physics/Dynamics/Subsystem ==
  Mechanism Configuration : sm_lib/Utilities/Mechanism Configuration  UniformGravity=Constant  GravityVector=[0 0 -9.80665]  GravityVectorUnits=m/s^2  LinearizationDelta=0.001  JointModeTransitionNonlinearIterations=2
  Rigid Transform : sm_lib/Frames and Transforms/Rigid Transform  RotationMethod=StandardAxis  FollAlignAxisA=+X  BaseAlignAxisA=+Y  FollAlignAxisB=+Y  BaseAlignAxisB=+Z  RotationStandardAxis=+X  RotationAngle=180  RotationAngleUnits=deg  RotationArbitraryAxis=[0 0 1]  RotationSequenceAxes=FollowerAxes  RotationSequence=XYX  RotationSequenceAngles=[0 0 0]  RotationSequenceAnglesUnits=deg  RotationMatrix=[1 0 0;0 1 0;0 0 1]  Quaternion=[1 0 0 0]  TranslationMethod=None  TranslationCartesianOffset=[0 0 0]  TranslationCartesianOffsetUnits=m  TranslationStandardAxis=+Z  TranslationStandardOffset=0  TranslationStandardOffsetUnits=m  TranslationROffset=0  TranslationROffsetUnits=m  TranslationThetaOffset=0  TranslationThetaOffsetUnits=deg  TranslationZOffset=0  TranslationZOffsetUnits=m
  Solver Configuration : nesl_utility/Solver Configuration  PhysicalDomain=network_engine_domain  SubClassName=solver  LeftPortType=input  RightPortType=generic  Tones=[]  Harmonics=[]  SimulateNoise=off  Profile=off  UseLocalSampling=off  EnableSwitchedLinearOptims=on  FrequencyDomain=off  UseCCode=off  RelTol=0.001  AbsTol=0.001  MinStep=1e-09  ToWorkspace=off  RevertToSquareIcSolve=off  NumHomotopyIterations=100  PhasorMode=off  PhasorModeNumHarmonics=1  ConsistencySolver=NEWTON_XTOL_AFTER_FTOL  IndexReductionMethod=DerivativeReplacement  DoDC=off  ResidualTolerance=1e-09  ConsistencyTolSource=GLOBAL  ConsistencyAbsTol=0.001  ConsistencyRelTol=0.001  ConsistencyTolFactor=0.001  UseLocalSolver=off  LocalSolverChoice=NE_BACKWARD_EULER_ADVANCER  ResolveIndetEquations=on  FunctionEvalNumThread=1  LocalSolverSampleTime=0.001  DoFixedCost=off  MaxNonlinIter=3  MaxModeIter=2  ComputeImpulses=off  ImpulseIterations=2  LinearAlgebra=auto  LinearAlgebraNumThread=0  EquationFormulation=NE_TIME_EF  DelaysMemoryBudget=1024  AutomaticFiltering=on  FilteringTimeConstant=0.001  PartitionStorageMethod=AS_NEEDED  PartitionMemoryBudget=1024  PartitionMethod=ROBUST  MultibodyUseLocalSolver=on  MultibodyLocalSolverChoice=ODE2  MultibodyLocalSolverSampleTime=0.001
  World Frame : sm_lib/Frames and Transforms/World Frame
  NED : PMIOPort  Side=Right
  connections:
  Rigid Transform/RConn1 -- NED/RConn1
  Mechanism Configuration/RConn1 -- Rigid Transform/LConn1 -- World Frame/RConn1 -- Solver Configuration/RConn1

== system Kirov_physics/Dynamics/Subsystem1 ==
  surface_input(deg) : Inport
  Degrees to Radians : simulink_extras/Transformations/Degrees to Radians
  Discrete Derivative : simulink/Quick Insert/Discrete/Discrete Derivative  gainval=1.0  ICPrevScaledInput=0.0  OutMin=[]  OutMax=[]  OutDataType=fixdt(1, 16)  OutScaling=2^-10  DoSatur=off
  Discrete Derivative1 : simulink/Quick Insert/Discrete/Discrete Derivative  gainval=1.0  ICPrevScaledInput=0.0  OutMin=[]  OutMax=[]  OutDataType=fixdt(1, 16)  OutScaling=2^-10  DoSatur=off
  Simulink-PS Converter : nesl_utility/Simulink-PS Converter  PhysicalDomain=network_engine_domain  SubClassName=ps_input  LeftPortType=input  RightPortType=output  PseudoPeriodic=off  Frequencies=[]  NoiseDistribution=none  NoiseParameters=[]  Unit=rad  AffineConversion=off  FilteringAndDerivatives=provide  SimscapeFilterOrder=1  InputFilterTimeConstant=0.001  UdotUserProvided=2
  surface_output : PMIOPort  Side=Right
  wires:
  surface_input(deg)/1 -> Degrees to Radians/1
  Discrete Derivative/1 -> Discrete Derivative1/1, Simulink-PS Converter/2
  Discrete Derivative1/1 -> Simulink-PS Converter/3
  Degrees to Radians/1 -> Discrete Derivative/1, Simulink-PS Converter/1
  connections:
  Simulink-PS Converter/RConn1 -- surface_output/RConn1

== system Kirov_physics/Dynamics/Subsystem10 ==
  torque_input(Nm) : Inport
  Discrete Derivative : simulink/Quick Insert/Discrete/Discrete Derivative  gainval=1.0  ICPrevScaledInput=0.0  OutMin=[]  OutMax=[]  OutDataType=fixdt(1, 16)  OutScaling=2^-10  DoSatur=off
  Discrete Derivative1 : simulink/Quick Insert/Discrete/Discrete Derivative  gainval=1.0  ICPrevScaledInput=0.0  OutMin=[]  OutMax=[]  OutDataType=fixdt(1, 16)  OutScaling=2^-10  DoSatur=off
  Simulink-PS Converter : nesl_utility/Simulink-PS Converter  PhysicalDomain=network_engine_domain  SubClassName=ps_input  LeftPortType=input  RightPortType=output  PseudoPeriodic=off  Frequencies=[]  NoiseDistribution=none  NoiseParameters=[]  Unit=N*m  AffineConversion=off  FilteringAndDerivatives=provide  SimscapeFilterOrder=1  InputFilterTimeConstant=0.001  UdotUserProvided=2
  torque_output : PMIOPort  Side=Right
  wires:
  Discrete Derivative1/1 -> Simulink-PS Converter/3
  Discrete Derivative/1 -> Simulink-PS Converter/2, Discrete Derivative1/1
  torque_input(Nm)/1 -> Simulink-PS Converter/1, Discrete Derivative/1
  connections:
  Simulink-PS Converter/RConn1 -- torque_output/RConn1

== system Kirov_physics/Dynamics/Subsystem11 ==
  torque_input(Nm) : Inport
  Discrete Derivative : simulink/Quick Insert/Discrete/Discrete Derivative  gainval=1.0  ICPrevScaledInput=0.0  OutMin=[]  OutMax=[]  OutDataType=fixdt(1, 16)  OutScaling=2^-10  DoSatur=off
  Discrete Derivative1 : simulink/Quick Insert/Discrete/Discrete Derivative  gainval=1.0  ICPrevScaledInput=0.0  OutMin=[]  OutMax=[]  OutDataType=fixdt(1, 16)  OutScaling=2^-10  DoSatur=off
  Simulink-PS Converter : nesl_utility/Simulink-PS Converter  PhysicalDomain=network_engine_domain  SubClassName=ps_input  LeftPortType=input  RightPortType=output  PseudoPeriodic=off  Frequencies=[]  NoiseDistribution=none  NoiseParameters=[]  Unit=N*m  AffineConversion=off  FilteringAndDerivatives=provide  SimscapeFilterOrder=1  InputFilterTimeConstant=0.001  UdotUserProvided=2
  torque_output : PMIOPort  Side=Right
  wires:
  torque_input(Nm)/1 -> Discrete Derivative/1, Simulink-PS Converter/1
  Discrete Derivative/1 -> Discrete Derivative1/1, Simulink-PS Converter/2
  Discrete Derivative1/1 -> Simulink-PS Converter/3
  connections:
  Simulink-PS Converter/RConn1 -- torque_output/RConn1

== system Kirov_physics/Dynamics/Subsystem12 ==
  torque_input(Nm) : Inport
  Discrete Derivative : simulink/Quick Insert/Discrete/Discrete Derivative  gainval=1.0  ICPrevScaledInput=0.0  OutMin=[]  OutMax=[]  OutDataType=fixdt(1, 16)  OutScaling=2^-10  DoSatur=off
  Discrete Derivative1 : simulink/Quick Insert/Discrete/Discrete Derivative  gainval=1.0  ICPrevScaledInput=0.0  OutMin=[]  OutMax=[]  OutDataType=fixdt(1, 16)  OutScaling=2^-10  DoSatur=off
  Simulink-PS Converter : nesl_utility/Simulink-PS Converter  PhysicalDomain=network_engine_domain  SubClassName=ps_input  LeftPortType=input  RightPortType=output  PseudoPeriodic=off  Frequencies=[]  NoiseDistribution=none  NoiseParameters=[]  Unit=N*m  AffineConversion=off  FilteringAndDerivatives=provide  SimscapeFilterOrder=1  InputFilterTimeConstant=0.001  UdotUserProvided=2
  torque_output : PMIOPort  Side=Right
  wires:
  Discrete Derivative1/1 -> Simulink-PS Converter/3
  Discrete Derivative/1 -> Simulink-PS Converter/2, Discrete Derivative1/1
  torque_input(Nm)/1 -> Simulink-PS Converter/1, Discrete Derivative/1
  connections:
  Simulink-PS Converter/RConn1 -- torque_output/RConn1

== system Kirov_physics/Dynamics/Subsystem13 ==
  flap_input : Inport
  Degrees to Radians : simulink_extras/Transformations/Degrees to Radians
  Gain2 : Gain  Gain=441.5/1000
  Gain3 : Gain  Gain=441.5/1000
  Subsystem13 : Subsystem
  Subsystem14 : Subsystem
  Subsystem15 : Subsystem
  dx : Lookup_n-D  NumberOfTableDimensions=1  BreakpointsForDimension1=[0, 1, 2]  BeginIndexSearchUsingPreviousIndexResult=on  Table=[0, -0.08819099, -0.21471805,]  InterpMethod=Linear Lagrange  DiagnosticForOutOfRangeInput=Error  InternalRulePriority=Speed  RndMeth=Simplest
  dz : Lookup_n-D  NumberOfTableDimensions=1  BreakpointsForDimension1=[0, 1, 2]  BeginIndexSearchUsingPreviousIndexResult=on  Table=[0, -0.15522630, -0.34229435]  InterpMethod=Linear Lagrange  DiagnosticForOutOfRangeInput=Error  InternalRulePriority=Speed  RndMeth=Simplest
  theta : Lookup_n-D  NumberOfTableDimensions=1  BreakpointsForDimension1=[0, 1, 2]  BeginIndexSearchUsingPreviousIndexResult=on  Table=[0, -13.24214507, -29.45123844]  InterpMethod=Linear Lagrange  DiagnosticForOutOfRangeInput=Error  InternalRulePriority=Speed  RndMeth=Simplest
  delta_x : PMIOPort  Side=Right
  delta_y : PMIOPort  Port=2  Side=Right
  rot_z : PMIOPort  Port=3  Side=Right
  wires:
  dz/1 -> Gain3/1
  Gain2/1 -> Subsystem14/1(surface_input)
  Gain3/1 -> Subsystem13/1(surface_input)
  dx/1 -> Gain2/1
  Degrees to Radians/1 -> Subsystem15/1(surface_input)
  theta/1 -> Degrees to Radians/1
  flap_input/1 -> dz/1, dx/1, theta/1
  connections:
  rot_z/RConn1 -- Subsystem15/RConn1
  Subsystem13/RConn1 -- delta_y/RConn1
  Subsystem14/RConn1 -- delta_x/RConn1

== system Kirov_physics/Dynamics/Subsystem14 ==
  surface_input(deg) : Inport
  Degrees to Radians : simulink_extras/Transformations/Degrees to Radians
  Discrete Derivative : simulink/Quick Insert/Discrete/Discrete Derivative  gainval=1.0  ICPrevScaledInput=0.0  OutMin=[]  OutMax=[]  OutDataType=fixdt(1, 16)  OutScaling=2^-10  DoSatur=off
  Discrete Derivative1 : simulink/Quick Insert/Discrete/Discrete Derivative  gainval=1.0  ICPrevScaledInput=0.0  OutMin=[]  OutMax=[]  OutDataType=fixdt(1, 16)  OutScaling=2^-10  DoSatur=off
  Simulink-PS Converter : nesl_utility/Simulink-PS Converter  PhysicalDomain=network_engine_domain  SubClassName=ps_input  LeftPortType=input  RightPortType=output  PseudoPeriodic=off  Frequencies=[]  NoiseDistribution=none  NoiseParameters=[]  Unit=rad  AffineConversion=off  FilteringAndDerivatives=provide  SimscapeFilterOrder=1  InputFilterTimeConstant=0.001  UdotUserProvided=2
  surface_output : PMIOPort  Side=Right
  wires:
  surface_input(deg)/1 -> Degrees to Radians/1
  Discrete Derivative/1 -> Discrete Derivative1/1, Simulink-PS Converter/2
  Discrete Derivative1/1 -> Simulink-PS Converter/3
  Degrees to Radians/1 -> Discrete Derivative/1, Simulink-PS Converter/1
  connections:
  Simulink-PS Converter/RConn1 -- surface_output/RConn1

== system Kirov_physics/Dynamics/Subsystem15 ==
  surface_input(deg) : Inport
  Degrees to Radians : simulink_extras/Transformations/Degrees to Radians
  Discrete Derivative : simulink/Quick Insert/Discrete/Discrete Derivative  gainval=1.0  ICPrevScaledInput=0.0  OutMin=[]  OutMax=[]  OutDataType=fixdt(1, 16)  OutScaling=2^-10  DoSatur=off
  Discrete Derivative1 : simulink/Quick Insert/Discrete/Discrete Derivative  gainval=1.0  ICPrevScaledInput=0.0  OutMin=[]  OutMax=[]  OutDataType=fixdt(1, 16)  OutScaling=2^-10  DoSatur=off
  Simulink-PS Converter : nesl_utility/Simulink-PS Converter  PhysicalDomain=network_engine_domain  SubClassName=ps_input  LeftPortType=input  RightPortType=output  PseudoPeriodic=off  Frequencies=[]  NoiseDistribution=none  NoiseParameters=[]  Unit=rad  AffineConversion=off  FilteringAndDerivatives=provide  SimscapeFilterOrder=1  InputFilterTimeConstant=0.001  UdotUserProvided=2
  surface_output : PMIOPort  Side=Right
  wires:
  Degrees to Radians/1 -> Simulink-PS Converter/1, Discrete Derivative/1
  Discrete Derivative1/1 -> Simulink-PS Converter/3
  Discrete Derivative/1 -> Simulink-PS Converter/2, Discrete Derivative1/1
  surface_input(deg)/1 -> Degrees to Radians/1
  connections:
  Simulink-PS Converter/RConn1 -- surface_output/RConn1

== system Kirov_physics/Dynamics/Subsystem16 ==
  flap_input : Inport
  Degrees to Radians : simulink_extras/Transformations/Degrees to Radians
  Gain2 : Gain  Gain=441.5/1000
  Gain3 : Gain  Gain=441.5/1000
  Subsystem13 : Subsystem
  Subsystem14 : Subsystem
  Subsystem15 : Subsystem
  dx : Lookup_n-D  NumberOfTableDimensions=1  BreakpointsForDimension1=[0, 1, 2]  BeginIndexSearchUsingPreviousIndexResult=on  Table=[0, -0.08819099, -0.21471805,]  InterpMethod=Linear Lagrange  DiagnosticForOutOfRangeInput=Error  InternalRulePriority=Speed  RndMeth=Simplest
  dz : Lookup_n-D  NumberOfTableDimensions=1  BreakpointsForDimension1=[0, 1, 2]  BeginIndexSearchUsingPreviousIndexResult=on  Table=[0, -0.15522630, -0.34229435]  InterpMethod=Linear Lagrange  DiagnosticForOutOfRangeInput=Error  InternalRulePriority=Speed  RndMeth=Simplest
  theta : Lookup_n-D  NumberOfTableDimensions=1  BreakpointsForDimension1=[0, 1, 2]  BeginIndexSearchUsingPreviousIndexResult=on  Table=[0, -13.24214507, -29.45123844]  InterpMethod=Linear Lagrange  DiagnosticForOutOfRangeInput=Error  InternalRulePriority=Speed  RndMeth=Simplest
  delta_x : PMIOPort  Side=Right
  delta_y : PMIOPort  Port=2  Side=Right
  rot_z : PMIOPort  Port=3  Side=Right
  wires:
  flap_input/1 -> theta/1, dx/1, dz/1
  theta/1 -> Degrees to Radians/1
  Degrees to Radians/1 -> Subsystem15/1(surface_input)
  dx/1 -> Gain2/1
  Gain3/1 -> Subsystem13/1(surface_input)
  Gain2/1 -> Subsystem14/1(surface_input)
  dz/1 -> Gain3/1
  connections:
  Subsystem14/RConn1 -- delta_x/RConn1
  Subsystem13/RConn1 -- delta_y/RConn1
  rot_z/RConn1 -- Subsystem15/RConn1

== system Kirov_physics/Dynamics/Subsystem17 ==
  surface_input(deg) : Inport
  Degrees to Radians : simulink_extras/Transformations/Degrees to Radians
  Discrete Derivative : simulink/Quick Insert/Discrete/Discrete Derivative  gainval=1.0  ICPrevScaledInput=0.0  OutMin=[]  OutMax=[]  OutDataType=fixdt(1, 16)  OutScaling=2^-10  DoSatur=off
  Discrete Derivative1 : simulink/Quick Insert/Discrete/Discrete Derivative  gainval=1.0  ICPrevScaledInput=0.0  OutMin=[]  OutMax=[]  OutDataType=fixdt(1, 16)  OutScaling=2^-10  DoSatur=off
  Simulink-PS Converter : nesl_utility/Simulink-PS Converter  PhysicalDomain=network_engine_domain  SubClassName=ps_input  LeftPortType=input  RightPortType=output  PseudoPeriodic=off  Frequencies=[]  NoiseDistribution=none  NoiseParameters=[]  Unit=rad  AffineConversion=off  FilteringAndDerivatives=provide  SimscapeFilterOrder=1  InputFilterTimeConstant=0.001  UdotUserProvided=2
  surface_output : PMIOPort  Side=Right
  wires:
  Degrees to Radians/1 -> Simulink-PS Converter/1, Discrete Derivative/1
  Discrete Derivative1/1 -> Simulink-PS Converter/3
  Discrete Derivative/1 -> Simulink-PS Converter/2, Discrete Derivative1/1
  surface_input(deg)/1 -> Degrees to Radians/1
  connections:
  Simulink-PS Converter/RConn1 -- surface_output/RConn1

== system Kirov_physics/Dynamics/Subsystem18 ==
  surface_input(deg) : Inport
  Degrees to Radians : simulink_extras/Transformations/Degrees to Radians
  Discrete Derivative : simulink/Quick Insert/Discrete/Discrete Derivative  gainval=1.0  ICPrevScaledInput=0.0  OutMin=[]  OutMax=[]  OutDataType=fixdt(1, 16)  OutScaling=2^-10  DoSatur=off
  Discrete Derivative1 : simulink/Quick Insert/Discrete/Discrete Derivative  gainval=1.0  ICPrevScaledInput=0.0  OutMin=[]  OutMax=[]  OutDataType=fixdt(1, 16)  OutScaling=2^-10  DoSatur=off
  Simulink-PS Converter : nesl_utility/Simulink-PS Converter  PhysicalDomain=network_engine_domain  SubClassName=ps_input  LeftPortType=input  RightPortType=output  PseudoPeriodic=off  Frequencies=[]  NoiseDistribution=none  NoiseParameters=[]  Unit=rad  AffineConversion=off  FilteringAndDerivatives=provide  SimscapeFilterOrder=1  InputFilterTimeConstant=0.001  UdotUserProvided=2
  surface_output : PMIOPort  Side=Right
  wires:
  surface_input(deg)/1 -> Degrees to Radians/1
  Discrete Derivative/1 -> Discrete Derivative1/1, Simulink-PS Converter/2
  Discrete Derivative1/1 -> Simulink-PS Converter/3
  Degrees to Radians/1 -> Discrete Derivative/1, Simulink-PS Converter/1
  connections:
  Simulink-PS Converter/RConn1 -- surface_output/RConn1

== system Kirov_physics/Dynamics/Subsystem19 ==
  prop_rad : Inport
  Discrete Derivative : simulink/Quick Insert/Discrete/Discrete Derivative  gainval=1.0  ICPrevScaledInput=0.0  OutMin=[]  OutMax=[]  OutDataType=fixdt(1, 16)  OutScaling=2^-10  DoSatur=off
  Discrete Derivative1 : simulink/Quick Insert/Discrete/Discrete Derivative  gainval=1.0  ICPrevScaledInput=0.0  OutMin=[]  OutMax=[]  OutDataType=fixdt(1, 16)  OutScaling=2^-10  DoSatur=off
  Simulink-PS Converter : nesl_utility/Simulink-PS Converter  PhysicalDomain=network_engine_domain  SubClassName=ps_input  LeftPortType=input  RightPortType=output  PseudoPeriodic=off  Frequencies=[]  NoiseDistribution=none  NoiseParameters=[]  Unit=rad  AffineConversion=off  FilteringAndDerivatives=provide  SimscapeFilterOrder=1  InputFilterTimeConstant=0.001  UdotUserProvided=2
  prop_output : PMIOPort  Side=Right
  wires:
  prop_rad/1 -> Simulink-PS Converter/1, Discrete Derivative/1
  Discrete Derivative1/1 -> Simulink-PS Converter/3
  Discrete Derivative/1 -> Simulink-PS Converter/2, Discrete Derivative1/1
  connections:
  Simulink-PS Converter/RConn1 -- prop_output/RConn1
